simulink model "bmsreq_can_unpack"  (R2026b)
settings: Solver=VariableStepAuto
undefined symbols (not defined in the file or in its folder): P, Ts
libraries: simulink x5, svdutilitieslib x1
settings Model: Creator=aomar  LastModifiedBy=aomar

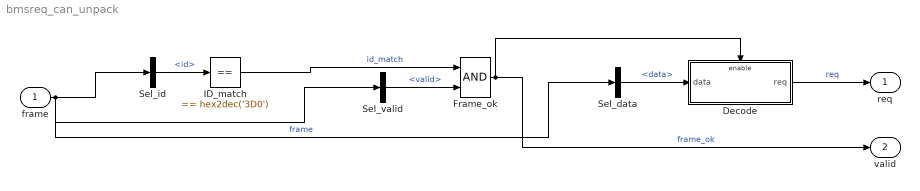
== system bmsreq_can_unpack ==
  frame : Inport  OutDataTypeStr=Bus: Bus_CanFrame8  SampleTime=Ts.can_slow
  Decode : Subsystem  TreatAsAtomicUnit=on
  Frame_ok : Logic  AllPortsSameDT=off  OutDataTypeStr=boolean
  ID_match : simulink/Logic and Bit Operations/Compare To Constant  relop===  const=hex2dec('3D0')  OutDataTypeStr=boolean
  Sel_data : BusSelector  OutputSignals=data
  Sel_id : BusSelector  OutputSignals=id
  Sel_valid : BusSelector  OutputSignals=valid
  req : Outport  OutDataTypeStr=Bus: Bus_BmsReq
  valid : Outport  Port=2  OutDataTypeStr=boolean
  wires:
  frame/1 -> Sel_id/1, Sel_data/1, Sel_valid/1  "frame"
  Sel_id/1 -> ID_match/1  "<id>"
  ID_match/1 -> Frame_ok/1  "id_match"
  Sel_valid/1 -> Frame_ok/2  "<valid>"
  Frame_ok/1 -> valid/1, Decode/Enable  "frame_ok"
  Sel_data/1 -> Decode/1(data)  "<data>"
  Decode/1(req) -> req/1  "req"

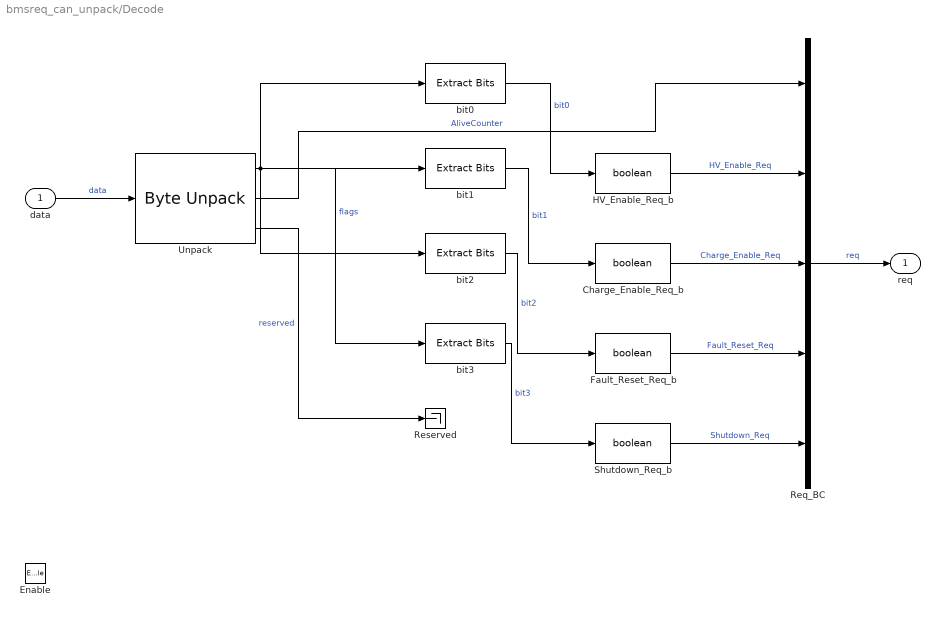
== system bmsreq_can_unpack/Decode ==
  data : Inport
  Enable : EnablePort
  Charge_Enable_Req_b : DataTypeConversion  OutDataTypeStr=boolean  SaturateOnIntegerOverflow=off  RndMeth=Floor
  Fault_Reset_Req_b : DataTypeConversion  OutDataTypeStr=boolean  SaturateOnIntegerOverflow=off  RndMeth=Floor
  HV_Enable_Req_b : DataTypeConversion  OutDataTypeStr=boolean  SaturateOnIntegerOverflow=off  RndMeth=Floor
  Req_BC : BusCreator  Inputs=5  OutDataTypeStr=Bus: Bus_BmsReq  NonVirtualBus=on
      settings: InheritFromInputs=off
  Reserved : Terminator
  Shutdown_Req_b : DataTypeConversion  OutDataTypeStr=boolean  SaturateOnIntegerOverflow=off  RndMeth=Floor
  Unpack : svdutilitieslib/Byte Unpack  dimensions={1,1,6}  datatypes={'uint8','uint8','uint8'}  byteAlign=1  blockPlatform=arduinoert
      settings: LibrarySourceBlock=mcblib/Signal Management/Byte Unpack
  bit0 : simulink/Logic and Bit Operations/Extract Bits  bitsToExtract=Range of bits  numBits=8  bitIdxRange=[0 0]  outScalingMode=Treat bit field as an integer
  bit1 : simulink/Logic and Bit Operations/Extract Bits  bitsToExtract=Range of bits  numBits=8  bitIdxRange=[1 1]  outScalingMode=Treat bit field as an integer
  bit2 : simulink/Logic and Bit Operations/Extract Bits  bitsToExtract=Range of bits  numBits=8  bitIdxRange=[2 2]  outScalingMode=Treat bit field as an integer
  bit3 : simulink/Logic and Bit Operations/Extract Bits  bitsToExtract=Range of bits  numBits=8  bitIdxRange=[3 3]  outScalingMode=Treat bit field as an integer
  req : Outport  OutDataTypeStr=Bus: Bus_BmsReq  InitialOutput=P.ic.Bus_BmsReq
  wires:
  data/1 -> Unpack/1  "data"
  Unpack/1 -> bit3/1, bit0/1, bit2/1, bit1/1  "flags"
  Unpack/2 -> Req_BC/1  "AliveCounter"
  Unpack/3 -> Reserved/1  "reserved"
  bit0/1 -> HV_Enable_Req_b/1  "bit0"
  bit1/1 -> Charge_Enable_Req_b/1  "bit1"
  bit2/1 -> Fault_Reset_Req_b/1  "bit2"
  bit3/1 -> Shutdown_Req_b/1  "bit3"
  HV_Enable_Req_b/1 -> Req_BC/2  "HV_Enable_Req"
  Charge_Enable_Req_b/1 -> Req_BC/3  "Charge_Enable_Req"
  Fault_Reset_Req_b/1 -> Req_BC/4  "Fault_Reset_Req"
  Shutdown_Req_b/1 -> Req_BC/5  "Shutdown_Req"
  Req_BC/1 -> req/1  "req"
